simulink model "MalhaAberta"  (R2024a)
settings: Solver=FixedStepDiscrete  StartTime=0.0  StopTime=Bancada.tRampa + Bancada.tRegime  FixedStep=Bancada.Tsim  RelTol=1e-3
undefined symbols (not defined in the file or in its folder): Bancada, DiscIntNeverNeededParam
libraries: spsDCVoltageSourceLib x2, spsVoltageMeasurementLib x2, spsThreePhaseSeriesRLCBranchLib x1, spsTwoLevelConverterLib x1, spsThreePhaseVIMeasurementLib x1, spsGroundLib x1, spspowerguiLib x1
settings Model: Creator=raphateixeira  LastModifiedBy=raphateixeira
settings DataIOCC: SaveOutput=off  SignalLogging=off  SaveTime=off
settings ConfigComp: CovBoundaryAbsTol=1.0e-5

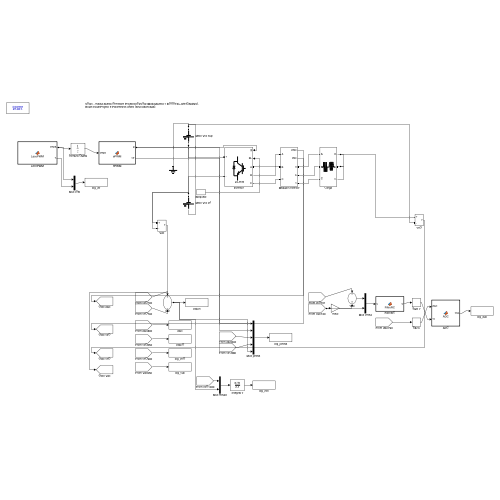
[thumbnail: Simulink's stored preview of the top-level diagram]
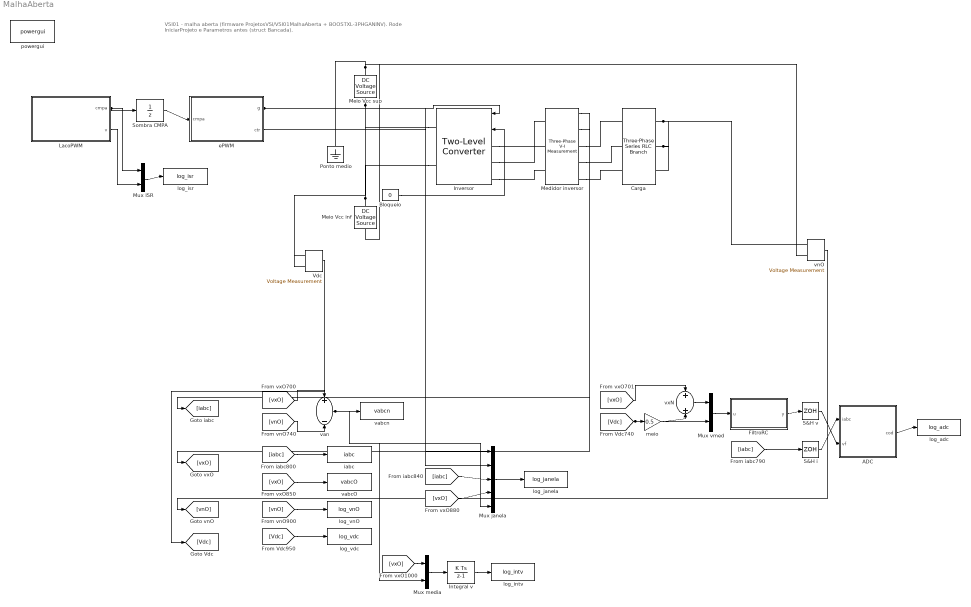
== system MalhaAberta ==
  note: VSI01 - malha aberta (firmware ProjetosVSI/VSI01MalhaAberta + BOOSTXL-3PHGANINV).
      | Rode IniciarProjeto e Parametros antes (struct Bancada).
  ADC : MATLAB Function  TreatAsAtomicUnit=on
  Bloqueio : Constant  Value=0
  Carga : spsThreePhaseSeriesRLCBranchLib/Three-Phase Series RLC Branch  LConnTagsString=A|B|C  RConnTagsString=A|B|C  BranchType=RL  Resistance=Bancada.RLf + Bancada.Rc  Inductance=Bancada.Lf  Capacitance=1e-6  Measurements=None
  FiltroRC : MATLAB Function  TreatAsAtomicUnit=on
  Integral v : DiscreteIntegrator  SampleTime=Bancada.Tsim  ICPrevOutput=DiscIntNeverNeededParam  ICPrevScaledInput=DiscIntNeverNeededParam
  Inversor : spsTwoLevelConverterLib/Two-Level Converter  ModelType=Switching function  Ron=Bancada.Ron  Rs=1e6  Cs=inf  Vforward=[0,0]  Ron_Diode=Bancada.Ron  Rs_Diode=1e6  Cs_Diode=inf  Vf_Diode=0  Rs_CurrentSource=inf  Ron_ACsource=1e-3
  LacoPWM : MATLAB Function  TreatAsAtomicUnit=on
  Medidor inversor : spsThreePhaseVIMeasurementLib/Three-Phase V-I Measurement  VoltageMeasurement=phase-to-ground  SetLabelV=off  LabelV=Vabc  Vpu=off  VpuLL=off  CurrentMeasurement=yes  SetLabelI=off  LabelI=Iabc  Ipu=off  Pbase=100e6  Vbase=500e3  OutputType=Complex  PhasorSimulation=off  PSBequivalent=0
  Meio Vcc inf : spsDCVoltageSourceLib/DC Voltage Source  Amplitude=Bancada.Vcc/2  Measurements=None
  Meio Vcc sup : spsDCVoltageSourceLib/DC Voltage Source  Amplitude=Bancada.Vcc/2  Measurements=None
  Mux ISR : Mux  Inputs=2
  Mux janela : Mux  Inputs=5
  Mux media : Mux  Inputs=2
  Mux vmed : Mux  Inputs=2
  Ponto medio : spsGroundLib/Ground  LConnTagsString=a
  S&H i : ZeroOrderHold  SampleTime=Bancada.Ts
  S&H v : ZeroOrderHold  SampleTime=Bancada.Ts
  Sombra CMPA : UnitDelay  InitialCondition=floor(Bancada.TBPRD/2)*ones(3,1)  SampleTime=Bancada.Ts  HasFrameUpgradeWarning=on
  Vdc : spsVoltageMeasurementLib/Voltage Measurement  PhasorSimulation=off  OutputType=Complex  PSBequivalent=0
  ePWM : MATLAB Function  TreatAsAtomicUnit=on
  iabc : ToWorkspace  VariableName=iabc  SaveFormat=Timeseries  SampleTime=Bancada.Tlog
  log_adc : ToWorkspace  VariableName=log_adc  SaveFormat=Timeseries  SampleTime=-1
  log_intv : ToWorkspace  VariableName=log_intv  SaveFormat=Timeseries  SampleTime=Bancada.Ts
  log_isr : ToWorkspace  VariableName=log_isr  SaveFormat=Timeseries  SampleTime=-1
  log_janela : ToWorkspace  VariableName=log_janela  SaveFormat=Timeseries  SampleTime=-1
      settings: MaxDataPoints=Bancada.nJanela
  log_vdc : ToWorkspace  VariableName=log_vdc  SaveFormat=Timeseries  SampleTime=Bancada.Tlog
  log_vnO : ToWorkspace  VariableName=log_vnO  SaveFormat=Timeseries  SampleTime=Bancada.Tlog
  meio : Gain  Gain=0.5
  powergui : spspowerguiLib/powergui  Priority=1  SimulationMode=Discrete  SampleTime=Bancada.Tsim  frequency=60  Iterations=50  frequencyindice=60  Pbase=100e6  ErrMax=1e-4  UnitsV=kV  UnitsW=MW  buscounter=0  FunctionMessages=off  echomessages=off  EnableUseOfTLC=off  CurrentSourceSwitches=off  DisableSnubberDevices=off  DisableRonSwitches=off  DisableVfSwitches=off  DisplayEquations=off  AutomaticDiscreteSolvers=off  SolverType=Tustin/Backward Euler (TBE)  Interpol=off  ExternalGateDelay=off  methode=off  Ts=100  x0status=blocks  SPID=on  SwTol=0  HookPort=off  NonlinearTolerance=1e-4  nMaxIteration=100  ContinueOnMaxIteration=off  RestoreLinks=warning  ResistiveCurrentMeasurement=off  Frange=[0:2:500]  Ylog=off  Xlog=on  ShowGrid=off  save=off  variable=ZData  structure=0  ZoomFFT=off  StartTime=0.0  cycles=1  DisplayStyle=1  fundamental=60  FreqAxis=off  MaxFrequency=1000  frequencyindicesteady=1  RmsSteady=1  display=off
  vabcO : ToWorkspace  VariableName=vabcO  SaveFormat=Timeseries  SampleTime=Bancada.Tlog
  vabcn : ToWorkspace  VariableName=vabcn  SaveFormat=Timeseries  SampleTime=Bancada.Tlog
  van : Sum  Inputs=+-
  vnO : spsVoltageMeasurementLib/Voltage Measurement  PhasorSimulation=off  OutputType=Complex  PSBequivalent=0
  vxN : Sum
  wires:
  LacoPWM/1(cmpa) -> Sombra CMPA/1, Mux ISR/1
  Sombra CMPA/1 -> ePWM/1(cmpa)
  ePWM/1(g) -> Inversor/1, Mux janela/1
  Bloqueio/1 -> Inversor/2
  Medidor inversor/2 -> [iabc]
  Medidor inversor/1 -> [vxO]
  vnO/1 -> [vnO]
  Vdc/1 -> [Vdc]
  [vxO] -> van/1
  [vnO] -> van/2
  [iabc] -> iabc/1
  [vxO] -> vabcO/1
  van/1 -> vabcn/1, Mux janela/5, Mux media/2
  [vnO] -> log_vnO/1
  [Vdc] -> log_vdc/1
  LacoPWM/2(v) -> Mux ISR/2
  Mux ISR/1 -> log_isr/1
  ePWM/2(ctr) -> Mux janela/2
  [iabc] -> Mux janela/3
  [vxO] -> Mux janela/4
  Mux janela/1 -> log_janela/1
  [vxO] -> Mux media/1
  Mux media/1 -> Integral v/1
  Integral v/1 -> log_intv/1
  [vxO] -> vxN/1
  [Vdc] -> meio/1, Mux vmed/2
  meio/1 -> vxN/2
  vxN/1 -> Mux vmed/1
  Mux vmed/1 -> FiltroRC/1(u)
  FiltroRC/1(y) -> S&H v/1
  [iabc] -> S&H i/1
  S&H i/1 -> ADC/1(iabc)
  S&H v/1 -> ADC/2(vf)
  ADC/1(cod) -> log_adc/1
  connections:
  Meio Vcc inf/RConn1 -- Meio Vcc sup/LConn1 -- Ponto medio/LConn1 -- vnO/LConn2
  Inversor/RConn1 -- Meio Vcc sup/RConn1 -- Vdc/LConn1
  Inversor/RConn2 -- Meio Vcc inf/LConn1 -- Vdc/LConn2
  Inversor/LConn1 -- Medidor inversor/LConn1
  Medidor inversor/RConn1 -- Carga/LConn1
  Inversor/LConn2 -- Medidor inversor/LConn2
  Medidor inversor/RConn2 -- Carga/LConn2
  Inversor/LConn3 -- Medidor inversor/LConn3
  Medidor inversor/RConn3 -- Carga/LConn3
  Carga/RConn2 -- Carga/RConn1 -- vnO/LConn1 -- Carga/RConn3

== matlab function MalhaAberta/LacoPWM ==
  settings: updateMethod=DISCRETE  sampleTime=Bancada.Ts
  data: cmpa output; v output; Bancada parameter
function [cmpa, v] = LacoPWM(Bancada)
% Laço do PWM (ISR do ePWM1, a cada Ts): espelho de senoides.c + PWM2v (placa.c) do
% firmware ProjetosCCS/ProjetosVSI/VSI01MalhaAberta, em float de 32 bits como no C28x.
%   v    = [va; vb; vc]: tensões de fase desejadas, em relação ao ponto médio do barramento [V]
%   cmpa = CMPA dos ePWM 1, 2, 3 (d = 1/2 + v/Vcc, limitada a 0..1, truncada como no cast do C)
persistent theta kRampa
if isempty(theta)
    theta = single(0);
    kRampa = uint32(0);
end
DOIS_PI   = single(6.283185307);
DOIS_PI_3 = single(2.094395102);
Ts     = single(1)/single(Bancada.fPWM);
Vcc    = single(Bancada.Vcc);
Vp     = min(single(Bancada.Vp), Vcc/single(2));        % sem sobremodulação
dTheta = DOIS_PI*single(Bancada.f)*Ts;
nRampa = uint32(floor(single(Bancada.tRampa)/Ts + single(0.5)));
periodo = single(Bancada.TBPRD);

% Senoides()
V = Vp;
if kRampa < nRampa
    V = Vp*single(kRampa)/single(nRampa);
    kRampa = kRampa + uint32(1);
end
vs = [V*sin(theta); V*sin(theta - DOIS_PI_3); V*sin(theta + DOIS_PI_3)];
theta = theta + dTheta;
if theta >= DOIS_PI
    theta = theta - DOIS_PI;
end

% PWM2v()
d = single(0.5) + vs/Vcc;
d = min(max(d, single(0)), single(1));
cmpa = double(floor(d*periodo));
v = double(vs);

== matlab function MalhaAberta/FiltroRC ==
  settings: updateMethod=DISCRETE  sampleTime=Bancada.Tsim
  data: u input; y output; Bancada parameter
function y = FiltroRC(u, Bancada)
% Filtro RC de 1a ordem das tensões medidas pelo BOOSTXL (VA, VB, VC, VDC), polo em fpTensao,
% discretizado por invariância ao degrau no passo Tsim.
persistent x
if isempty(x)
    x = zeros(4,1);
end
a = 1 - exp(-2*pi*Bancada.fpTensao*Bancada.Tsim);
x = x + a*(u - x);
y = x;

== matlab function MalhaAberta/ADC ==
  data: iabc input; cod output; vf input; Bancada parameter
function cod = ADC(iabc, vf, Bancada)
% Códigos do ADC (12 bits, 0 a 3,3 V) das medidas do BOOSTXL-3PHGANINV, amostradas em CTR = 0:
%  - correntes de fase: shunt em linha de 5 mohm + INA240 (ganho 20), ponto médio 1,65 V e
%    polaridade invertida (USER_M1_SIGN_CURRENT_SF = -1 no SDK): v = 1,65 - 0,1 i  (+-16,5 A)
%  - VA, VB, VC (em relação ao negativo do barramento) e VDC: divisor com fundo de escala de
%    81,5 V, já filtradas pelo RC (bloco FiltroRC)
%   cod = [IA; IB; IC; VA; VB; VC; VDC]
vi = Bancada.Vmeio - Bancada.Gina*Bancada.Rsh*iabc(:);
vv = vf(:)*Bancada.Vadc/Bancada.VfsTensao;
n = 2^Bancada.nbits;
cod = min(max(floor([vi; vv]/Bancada.Vadc*n), 0), n - 1);

== matlab function MalhaAberta/ePWM ==
  settings: updateMethod=DISCRETE  sampleTime=Bancada.Tsim
  data: cmpa input; g output; ctr output; Bancada parameter
function [g, ctr] = ePWM(cmpa, Bancada)
% ePWM 1, 2, 3 do F28379D configurados como em placa.c (VSI01), emulados contagem a contagem:
%  - contador sobe e desce, 0 -> TBPRD -> 0 (período 2*TBPRD contagens de EPWMCLK);
%  - CMPA com sombra: o valor escrito pela ISR só vale a partir do próximo CTR = 0;
%  - AQ: saída A vai a 0 em CTR = CMPA subindo e a 1 em CTR = CMPA descendo;
%  - banda morta: EPWMxA = A com a subida atrasada de nMorto (RED);
%    EPWMxB = A invertida, com a subida atrasada de nMorto (FED, polaridade ativa baixa).
% Cada passo de Tsim avança k = Tsim*EPWMCLK contagens; os eventos caem no primeiro passo
% em que o contador cruza CMPA (erro de até k-1 contagens).
%   g   = [AH AL BH BL CH CL]: comando das chaves (1 = ligada)
%   ctr = TBCTR do ePWM1
persistent pos A desde ativo
P   = round(Bancada.TBPRD);
k   = round(Bancada.Tsim*Bancada.EPWMCLK);
nDB = round(Bancada.tMorto*Bancada.EPWMCLK);
if isempty(pos)
    pos = -1;                    % primeira chamada: estado inicial em t = 0
    A = false(3,1);              % AQ parte com a saída A em 0
    desde = nDB*ones(3,1);       % contagens desde a última transição de A
    ativo = floor(P/2)*ones(3,1);   % CMPA inicial (d = 1/2)
end
if pos < 0
    pos = 0;
    ctrAnt = 0;
    subindo = true;
else
    ctrAnt = pos;
    if pos > P
        ctrAnt = 2*P - pos;
    end
    subindo = pos < P;
    pos = mod(pos + k, 2*P);
end
ctr = pos;
if pos > P
    ctr = 2*P - pos;
end
for i = 1:3
    C = ativo(i);
    if subindo && ctrAnt < C && ctr >= C && A(i)
        A(i) = false;
        desde(i) = ctr - C;
    elseif ~subindo && ctrAnt > C && ctr <= C && ~A(i)
        A(i) = true;
        desde(i) = C - ctr;
    else
        desde(i) = desde(i) + k;
    end
end
if pos == 0
    ativo = cmpa(:);             % carga da sombra em CTR = 0
end
g = zeros(6,1);
for i = 1:3
    passou = desde(i) >= nDB;
    g(2*i-1) = double(A(i) && passou);
    g(2*i)   = double(~A(i) && passou);
end
